simulink model "imuCal"  (Simulink 9.0)
settings: Solver=FixedStepAuto  StartTime=0.0  StopTime=10.0  RelTol=1e-3
libraries: lib_imuCal x1
settings Model: Creator=currisd  LastModifiedBy=CurriSD
settings DataIOCC: SaveFormat=Dataset
settings OptimizationCC: DefaultParameterBehavior=Inlined  PassReuseOutputArgsAs=Individual arguments  LifeSpan=auto
settings DebuggingCC: UnderspecifiedInitializationDetection=Simplified  MergeDetectMultiDrivingBlocksExec=error  ParameterTunabilityLossMsg=error  SFUnexpectedBacktrackingDiag=error  SFNoUnconditionalDefaultTransitionDiag=error  SFExecutionAtInitializationDiag=warning
settings HardwareCC: ProdBitPerPointer=64  ProdBitPerSizeT=64  ProdBitPerPtrDiffT=64  ProdLargestAtomicFloat=Float  ProdIntDivRoundTo=Zero  ProdEndianess=LittleEndian  ProdWordSize=64  ProdHWDeviceType=Intel->x86-64 (Windows64)
settings ModelReferenceCC: PropagateSignalLabelsOutOfModel=on
settings SFSimCC: MATLABDynamicMemAlloc=off
settings RTWCC: SystemTargetFile=ert.tlc  GenCodeOnly=on  TemplateMakefile=ert_default_tmf  Description=Embedded Coder  GenerateReport=on  IncludeHyperlinkInReport=on  LaunchReport=on  GenerateTraceInfo=on  GenerateTraceReport=on  GenerateTraceReportSl=on  GenerateTraceReportSf=on  GenerateTraceReportEml=on
settings CodeAppCC: ForceParamTrailComments=on  IgnoreCustomStorageClasses=off  OperatorAnnotations=on  SimulinkDataObjDesc=on  SFDataObjDesc=on  InsertBlockDesc=on  StateflowObjectComments=off
settings ERTTargetCC: TargetLangStandard=C99 (ISO)  GenerateSampleERTMain=on  MultiInstanceERTCode=on  CodeInterfacePackaging=Reusable function  SupportVariableSizeSignals=on  InlinedParameterPlacement=NonHierarchical  RootIOFormat=Part of model data structure  ERTCustomFileTemplate=example_file_process.tlc
settings ConfigComp: CovMetricSettings=dwe  CovHtmlReporting=off  CovSaveCumulativeToWorkspaceVar=off  CovSaveSingleToWorkspaceVar=off  CovExternalEMLEnable=on

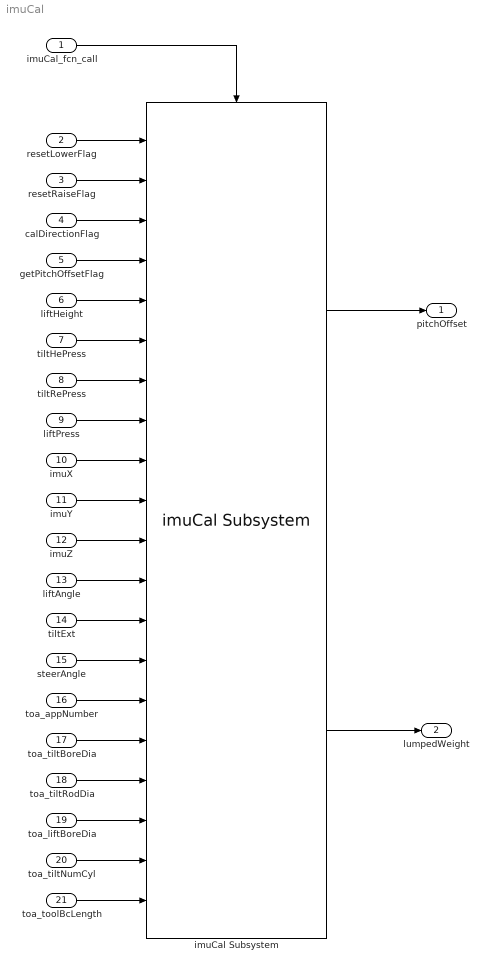
== system imuCal ==
  imuCal_fcn_call : Inport  OutputFunctionCall=on
  resetLowerFlag : Inport  Port=2
  resetRaiseFlag : Inport  Port=3
  calDirectionFlag : Inport  Port=4
  getPitchOffsetFlag : Inport  Port=5
  liftHeight : Inport  Port=6
  tiltHePress : Inport  Port=7
  tiltRePress : Inport  Port=8
  liftPress : Inport  Port=9
  imuX : Inport  Port=10
  imuY : Inport  Port=11
  imuZ : Inport  Port=12
  liftAngle : Inport  Port=13
  tiltExt : Inport  Port=14
  steerAngle : Inport  Port=15
  toa_appNumber : Inport  Port=16  OutDataTypeStr=uint32
  toa_tiltBoreDia : Inport  Port=17  OutDataTypeStr=single
  toa_tiltRodDia : Inport  Port=18  OutDataTypeStr=single
  toa_liftBoreDia : Inport  Port=19  OutDataTypeStr=single
  toa_tiltNumCyl : Inport  Port=20  OutDataTypeStr=uint8
  toa_toolBcLength : Inport  Port=21  OutDataTypeStr=single
  imuCal Subsystem : lib_imuCal/imuCal Subsystem
  pitchOffset : Outport
  lumpedWeight : Outport  Port=2
  wires:
  imuCal_fcn_call/1 -> imuCal Subsystem/Trigger
  resetLowerFlag/1 -> imuCal Subsystem/1
  resetRaiseFlag/1 -> imuCal Subsystem/2
  calDirectionFlag/1 -> imuCal Subsystem/3
  getPitchOffsetFlag/1 -> imuCal Subsystem/4
  liftHeight/1 -> imuCal Subsystem/5
  tiltHePress/1 -> imuCal Subsystem/6
  tiltRePress/1 -> imuCal Subsystem/7
  liftPress/1 -> imuCal Subsystem/8
  imuX/1 -> imuCal Subsystem/9
  imuY/1 -> imuCal Subsystem/10
  imuZ/1 -> imuCal Subsystem/11
  liftAngle/1 -> imuCal Subsystem/12
  tiltExt/1 -> imuCal Subsystem/13
  steerAngle/1 -> imuCal Subsystem/14
  imuCal Subsystem/1 -> pitchOffset/1
  toa_appNumber/1 -> imuCal Subsystem/15
  toa_tiltBoreDia/1 -> imuCal Subsystem/16
  toa_tiltRodDia/1 -> imuCal Subsystem/17
  toa_liftBoreDia/1 -> imuCal Subsystem/18
  toa_tiltNumCyl/1 -> imuCal Subsystem/19
  toa_toolBcLength/1 -> imuCal Subsystem/20
  imuCal Subsystem/2 -> lumpedWeight/1
